simulink model "ur5_gravity_probe"  (R2024b)
settings: Solver=ode4  StartTime=0.0  StopTime=1  FixedStep=0.001  RelTol=1e-3
undefined symbols (not defined in the file): dq0_ur5, gc_on_ur5, q0_ur5
libraries: robotmaniplib x2
settings Model: Creator=ENVY  LastModifiedBy=ENVY

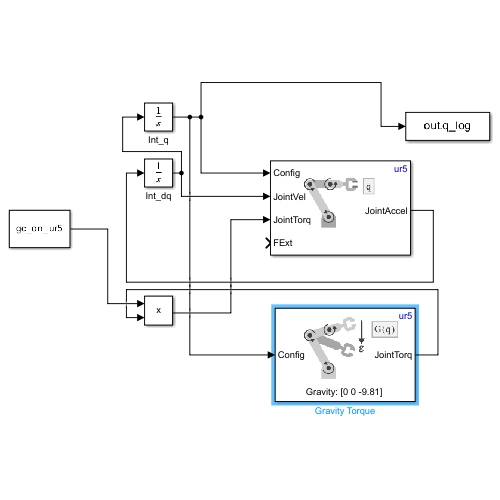
[thumbnail: Simulink's stored preview of the top-level diagram]
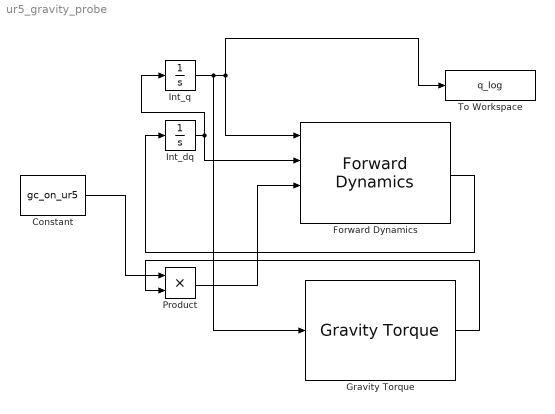
== system ur5_gravity_probe ==
  Constant : Constant  Value=gc_on_ur5
  Forward Dynamics : robotmaniplib/Forward Dynamics  RigidBodyTree=ur5  SimulateUsing=Interpreted execution
  Gravity Torque : robotmaniplib/Gravity Torque  RigidBodyTree=ur5  SimulateUsing=Interpreted execution
  Int_dq : Integrator  InitialCondition=dq0_ur5
  Int_q : Integrator  InitialCondition=q0_ur5
  Product : Product
  To Workspace : ToWorkspace  VariableName=q_log  SampleTime=-1
      settings: Save2DSignal=2-D array (concatenate along first dimension)
  wires:
  Constant/1 -> Product/1
  Int_q/1 -> To Workspace/1, Forward Dynamics/1, Gravity Torque/1
  Int_dq/1 -> Int_q/1, Forward Dynamics/2
  Gravity Torque/1 -> Product/2
  Product/1 -> Forward Dynamics/3
  Forward Dynamics/1 -> Int_dq/1
